simulink model "ex9_led"  (Simulink 7.6)
settings: Solver=FixedStepDiscrete  SolverMode=SingleTasking  StartTime=0.0  StopTime=inf  FixedStep=0.001  RelTol=1e-3
libraries: dsPICdrivers x9, simulink x5
settings Model: Creator=Lior  LastModifiedBy=Lior  BufferReuse=off
settings OptimizationCC: BlockReduction=off  InlineParams=on  BufferReuse=off  OptimizeModelRefInitCode=on  LifeSpan=1
settings HardwareCC: ProdBitPerInt=16  ProdBitPerPointer=16  ProdEndianess=LittleEndian  ProdWordSize=16  ProdHWDeviceType=16-bit Generic
settings RTWCC: SystemTargetFile=dspic.tlc  MakeCommand=make_CreateMPLAB  TemplateMakefile=dspic_pic30_gcc.tmf  PostCodeGenCommand=dsPIC_Compile()  Description=Embedded Target for Microchip dsPIC (real-time)  ProcessScript=dspic_make_rtw_hook
settings CodeAppCC: IgnoreCustomStorageClasses=off
settings STFCustomTargetCC: IncludeMdlTerminateFcn=off  CombineOutputUpdateFcns=on  SuppressErrorStatus=on  ERTCustomFileBanners=on  SupportContinuousTime=off  SupportNonInlinedSFcns=off  SystemTargetFile=dspic.tlc
settings ERTTargetCC: MultiwordLength=2048  ParMdlRefBuildCompliant=off  CompOptLevelCompliant=off  IncludeMdlTerminateFcn=off  SuppressErrorStatus=on  ERTFirstTimeCompliant=off  ModelStepFunctionPrototypeControlCompliant=off  CPPClassGenCompliant=off  ExtModeMexFile=ext_serial_win32_comm  InlinedParameterPlacement=NonHierarchical  ERTSrcFileBannerTemplate=dsPIC_code_template.cgt  ERTHdrFileBannerTemplate=dsPIC_code_template.cgt  ERTDataSrcFileTemplate=dsPIC_code_template.cgt  ERTDataHdrFileTemplate=dsPIC_code_template.cgt  ERTCustomFileTemplate=dsPIC_main.tlc  ConvertIfToSwitch=off
settings CustomProperty: DataType=string  Value=C:\PROGRA~1\MATLAB\R2010b\bin\win64\gmake

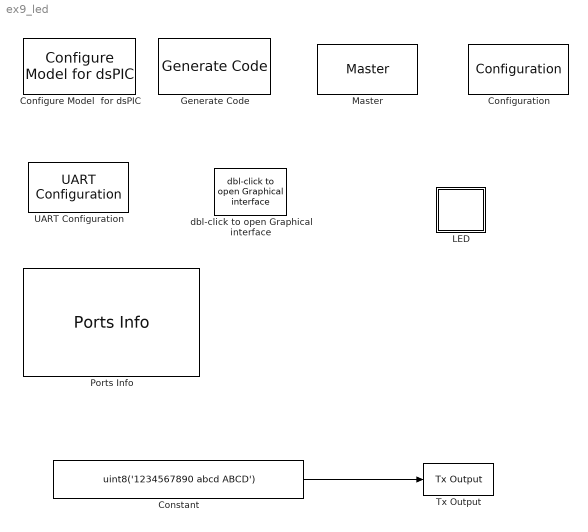
== system ex9_led ==
  Configuration : dsPICdrivers/Configuration  SystemSampleTime=-1  double64=off
  Configure Model  for dsPIC : dsPICdrivers/Simulink Configuration/Configure Model  for dsPIC
  Constant : Constant  Value=uint8('1234567890 abcd ABCD')  OutDataTypeStr=uint8  SampleTime=0.1
  Generate Code : dsPICdrivers/Simulink Configuration/Generate Code
  LED : Subsystem
  Master : dsPICdrivers/Master  Tag=dsPIC_MASTER  Priority=1  TimeStepType=Timer1  picType=33fJ256GP710  fcy=6250000  Quartz_33f=14e6  PLLActive_33f=on  fcyDesired_33f=0  tmr1="[1  6249  0]"  tmr1Info="Time Step : 0.001  ;   Error : 0%  PR1=6249"  tmr2345="[0  0  0  0  0  0  0  0]"  tmr2345cfg=[-1 -1 -1 -1 -1 -1 -1 -1]  IOautoConf=on  typePort="[ 0   0   0   0   0   0   0   0   0   0   0   0   0   0   0   0   0   0   0   0   0   0   0   0   0   0   0   0   0   0   0   0   0   0   0   0   0   0   0   0   0   0   0   0   0   0   0   0   0   0   0   0   0   0   0   0   0   0   0   0   0   0   0   0   0  10  10  10  10   0   0   0   0   0   0   0   0   0   0   0   0   0   0   0   4   5   0   0   0   0   0   0   0   0   0   0   0   0   0   0   0   0   0   0   0   0   0   0   0   0   0   0 ]"  TRIS="[ 65535  65535  65535  65535  65505  65535  65535 ]"  ADPCFG=503316480  MasterBusyPort=None  MasterOverloadPort=None  FOSC=Quartz (XT - HS)  ClockSwitchMonitor=Both disabled  TempProtection_33f=TEMP_ON  FPBOR=<empty>  PWRT=disable  MCLR=<empty>  ICD=ICS_PGD1  JTAGEN=JTAGEN_OFF  PowerSave=off  OverrideFcy=off  NewFcy=1e6  PR2345="[65535  65535  65535  65535  65535  65535  65535  65535]"
  Ports Info : dsPICdrivers/Ports Info  Tag=dsPIC_PortInfo
  Tx Output : dsPICdrivers/Serial PORT/Tx Output  Tag=dsPIC_TX  Priority=5  UART=2  OrderingInOutPopup=None
  UART Configuration : dsPICdrivers/Serial PORT/UART Configuration  Tag=dsPIC_config_UART  Priority=2  UART=2  proposed_BAUD=Custom  BAUD=202700  ALT_TX_RX=on  InterruptTxWhen=When Transmit Buffer is empty  TXInterruptPri=1  TxBufferSize=32  TXEN=on  InterruptRxWhen=When Receive Buffer is full (contain 4 characters)  RXInterruptPri=2  RxBufferSize=32  DoNotImplementRxInterrupt=off  DoNotImplementTxInterrupt=off  UxBRG=1  Info="UxBRG = 1   ||  Real Baud : 195313   ||  % error : -3.6445  ||  max 19.5313 Bytes / Step"  RealBaud=0  ERROR=-3.6445  BYTES_STEP=19.5313
  dbl-click to open Graphical interface : dsPICdrivers/Serial PORT/dbl-click to open Graphical interface  Nothing=0
  wires:
  Constant/1 -> Tx Output/1

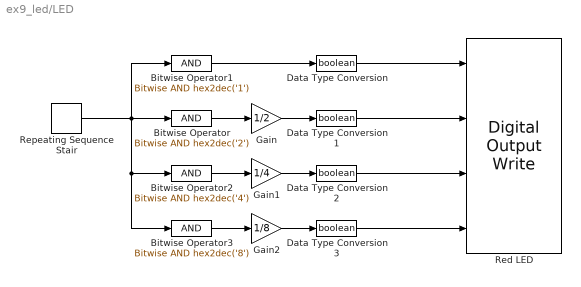
== system ex9_led/LED ==
  Bitwise Operator : simulink/Logic and Bit Operations/Bitwise Operator  logicop=AND  UseBitMask=on  BitMask=hex2dec('2')  BitMaskRealWorld=Stored Integer
  Bitwise Operator1 : simulink/Logic and Bit Operations/Bitwise Operator  logicop=AND  UseBitMask=on  BitMask=hex2dec('1')  BitMaskRealWorld=Stored Integer
  Bitwise Operator2 : simulink/Logic and Bit Operations/Bitwise Operator  logicop=AND  UseBitMask=on  BitMask=hex2dec('4')  BitMaskRealWorld=Stored Integer
  Bitwise Operator3 : simulink/Logic and Bit Operations/Bitwise Operator  logicop=AND  UseBitMask=on  BitMask=hex2dec('8')  BitMaskRealWorld=Stored Integer
  Data Type Conversion{,1..3} (4 alike) : DataTypeConversion  OutDataTypeStr=boolean
  Gain : Gain  Gain=1/2
  Gain1 : Gain  Gain=1/4
  Gain2 : Gain  Gain=1/8
  Red LED : dsPICdrivers/Digital I//O/Digital Output Write  Tag=dsPIC_Digital_Output  Priority=5  PORT=E  Pin=[1 2 3 4]  Simultaneous=on  OrderingInOutPopup=None
  Repeating Sequence Stair : simulink/Sources/Repeating Sequence Stair  SystemSampleTime=-1  OutValues=[1:15].'  tsamp=0.1  OutMin=[]  OutMax=[]  OutDataTypeStr=uint8  OutputDataTypeScalingMode=uint8  OutDataType=fixdt(0,8)  ConRadixGroup=Best Precision: Vector-wise  OutScaling=2^-12
  wires:
  Data Type Conversion/1 -> Red LED/1
  Data Type Conversion1/1 -> Red LED/2
  Data Type Conversion2/1 -> Red LED/3
  Data Type Conversion3/1 -> Red LED/4
  Bitwise Operator1/1 -> Data Type Conversion/1
  Bitwise Operator/1 -> Gain/1
  Bitwise Operator2/1 -> Gain1/1
  Bitwise Operator3/1 -> Gain2/1
  Repeating Sequence Stair/1 -> Bitwise Operator/1, Bitwise Operator1/1, Bitwise Operator2/1, Bitwise Operator3/1
  Gain/1 -> Data Type Conversion1/1
  Gain1/1 -> Data Type Conversion2/1
  Gain2/1 -> Data Type Conversion3/1
